simulink model "speed_pi_float"  (R2026b)
settings: Solver=FixedStepDiscrete  StopTime=0.01  FixedStep=0.0001
model workspace (MAT data in the model file):
  Iq_int_limit = 0.5
  Kaw_s = 0.08
  Ki_ASR = 1.44267798821
  Kp_ASR = 0.0180334748527
  Speed_loop_Iq_Limit = 1
  Ts = 0.0001
  Ts_ASR = 0.001
  v_ff_eps = 0.5
  v_over_eps = 3
  v_ref_zero_eps = 0
settings Model: Creator=lww  LastModifiedBy=lww

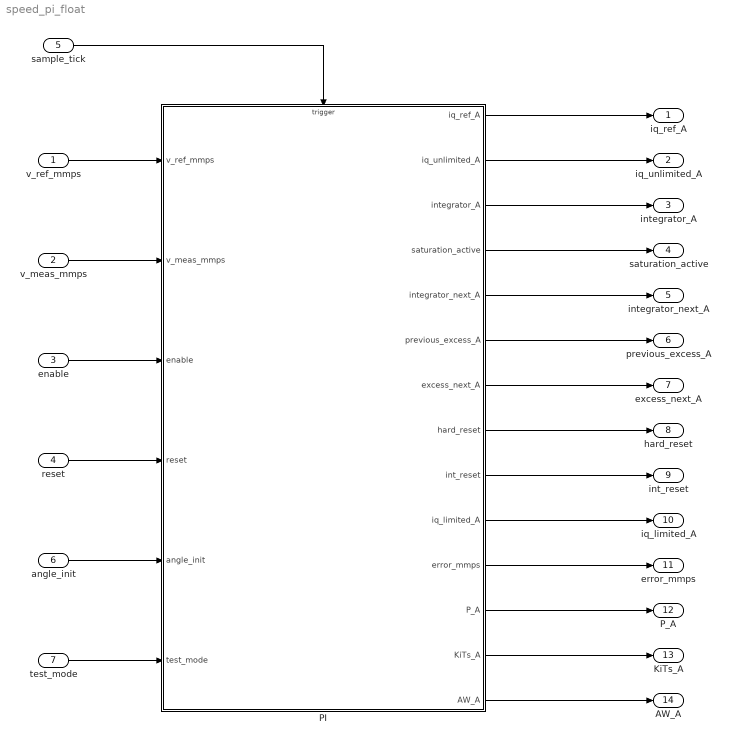
== system speed_pi_float ==
  v_ref_mmps : Inport
  v_meas_mmps : Inport  Port=2
  enable : Inport  Port=3
  reset : Inport  Port=4
  sample_tick : Inport  Port=5
  angle_init : Inport  Port=6
  test_mode : Inport  Port=7
  PI : Subsystem
  iq_ref_A : Outport
  iq_unlimited_A : Outport  Port=2
  integrator_A : Outport  Port=3
  saturation_active : Outport  Port=4
  integrator_next_A : Outport  Port=5
  previous_excess_A : Outport  Port=6
  excess_next_A : Outport  Port=7
  hard_reset : Outport  Port=8
  int_reset : Outport  Port=9
  iq_limited_A : Outport  Port=10
  error_mmps : Outport  Port=11
  P_A : Outport  Port=12
  KiTs_A : Outport  Port=13
  AW_A : Outport  Port=14
  wires:
  v_ref_mmps/1 -> PI/1(v_ref_mmps)
  sample_tick/1 -> PI/Trigger
  angle_init/1 -> PI/5(angle_init)
  v_meas_mmps/1 -> PI/2(v_meas_mmps)
  test_mode/1 -> PI/6(test_mode)
  enable/1 -> PI/3(enable)
  reset/1 -> PI/4(reset)
  PI/1(iq_ref_A) -> iq_ref_A/1
  PI/2(iq_unlimited_A) -> iq_unlimited_A/1
  PI/3(integrator_A) -> integrator_A/1
  PI/4(saturation_active) -> saturation_active/1
  PI/5(integrator_next_A) -> integrator_next_A/1
  PI/6(previous_excess_A) -> previous_excess_A/1
  PI/7(excess_next_A) -> excess_next_A/1
  PI/8(hard_reset) -> hard_reset/1
  PI/9(int_reset) -> int_reset/1
  PI/10(iq_limited_A) -> iq_limited_A/1
  PI/11(error_mmps) -> error_mmps/1
  PI/12(P_A) -> P_A/1
  PI/13(KiTs_A) -> KiTs_A/1
  PI/14(AW_A) -> AW_A/1

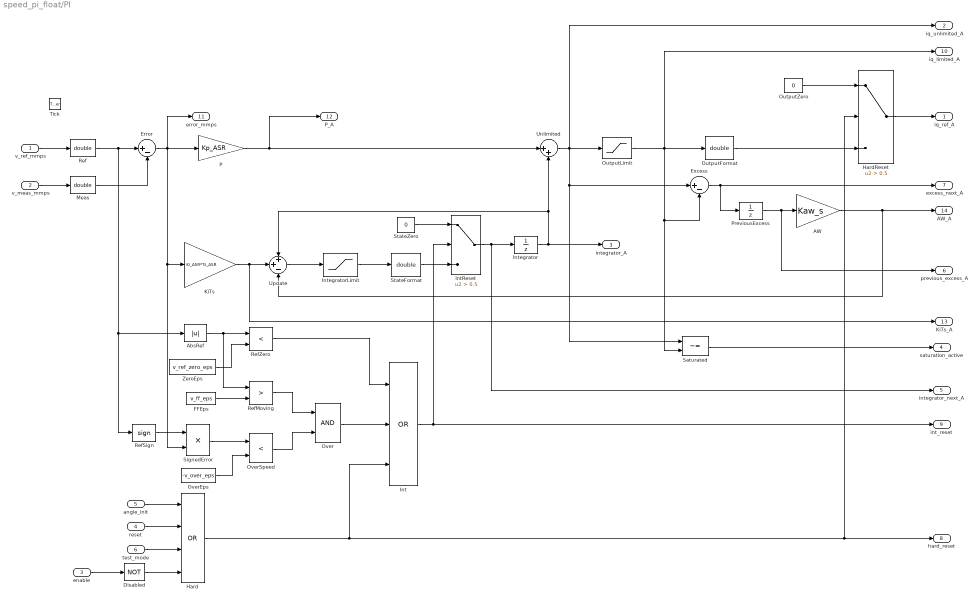
== system speed_pi_float/PI ==
  v_ref_mmps : Inport
  v_meas_mmps : Inport  Port=2
  enable : Inport  Port=3
  reset : Inport  Port=4
  angle_init : Inport  Port=5
  test_mode : Inport  Port=6
  Tick : TriggerPort  VariantControl=(inherit)
  AW : Gain  Gain=Kaw_s  ParamDataTypeStr=double  OutDataTypeStr=double  RndMeth=Convergent  SaturateOnIntegerOverflow=on
  AbsRef : Abs  RndMeth=Convergent
  Disabled : Logic  Operator=NOT  AllPortsSameDT=off  OutDataTypeStr=boolean
  Error : Sum  Inputs=|+-  OutDataTypeStr=double  AccumDataTypeStr=double  RndMeth=Convergent  SaturateOnIntegerOverflow=on
  Excess : Sum  Inputs=|+-  OutDataTypeStr=double  AccumDataTypeStr=double  RndMeth=Convergent  SaturateOnIntegerOverflow=on
  FFEps : Constant  Value=v_ff_eps  OutDataTypeStr=double
  Hard : Logic  Operator=OR  Inputs=4  AllPortsSameDT=off  OutDataTypeStr=boolean
  HardReset : Switch  Criteria=u2 > Threshold  Threshold=0.5  RndMeth=Convergent  InputSameDT=off
  Int : Logic  Operator=OR  Inputs=3  AllPortsSameDT=off  OutDataTypeStr=boolean
  IntReset : Switch  Criteria=u2 > Threshold  Threshold=0.5  RndMeth=Convergent  InputSameDT=off
  Integrator : UnitDelay  SampleTime=-1
  IntegratorLimit : Saturate  UpperLimit=Iq_int_limit  LowerLimit=-Iq_int_limit  RndMeth=Convergent
  KiTs : Gain  Gain=Ki_ASR*Ts_ASR  ParamDataTypeStr=double  OutDataTypeStr=double  RndMeth=Convergent  SaturateOnIntegerOverflow=on
  Meas : DataTypeConversion  OutDataTypeStr=double  RndMeth=Convergent
  OutputFormat : DataTypeConversion  OutDataTypeStr=double  RndMeth=Convergent
  OutputLimit : Saturate  UpperLimit=Speed_loop_Iq_Limit  LowerLimit=-Speed_loop_Iq_Limit  RndMeth=Convergent
  OutputZero : Constant  Value=0  OutDataTypeStr=double
  Over : Logic  AllPortsSameDT=off  OutDataTypeStr=boolean
  OverEps : Constant  Value=-v_over_eps  OutDataTypeStr=double
  OverSpeed : RelationalOperator  Operator=<  RndMeth=Convergent  InputSameDT=off
  P : Gain  Gain=Kp_ASR  ParamDataTypeStr=double  OutDataTypeStr=double  RndMeth=Convergent  SaturateOnIntegerOverflow=on
  PreviousExcess : UnitDelay  SampleTime=-1
  Ref : DataTypeConversion  OutDataTypeStr=double  RndMeth=Convergent
  RefMoving : RelationalOperator  Operator=>  RndMeth=Convergent  InputSameDT=off
  RefSign : Signum
  RefZero : RelationalOperator  Operator=<  RndMeth=Convergent  InputSameDT=off
  Saturated : RelationalOperator  Operator=~=  RndMeth=Convergent  InputSameDT=off
  SignedError : Product  OutDataTypeStr=double  RndMeth=Convergent  SaturateOnIntegerOverflow=on
  StateFormat : DataTypeConversion  OutDataTypeStr=double  RndMeth=Convergent
  StateZero : Constant  Value=0  OutDataTypeStr=double
  Unlimited : Sum  Inputs=|++  OutDataTypeStr=double  AccumDataTypeStr=double  RndMeth=Convergent  SaturateOnIntegerOverflow=on
  Update : Sum  Inputs=++-  OutDataTypeStr=double  AccumDataTypeStr=double  RndMeth=Convergent  SaturateOnIntegerOverflow=on
  ZeroEps : Constant  Value=v_ref_zero_eps  OutDataTypeStr=double
  iq_ref_A : Outport
  iq_unlimited_A : Outport  Port=2
  integrator_A : Outport  Port=3
  saturation_active : Outport  Port=4
  integrator_next_A : Outport  Port=5
  previous_excess_A : Outport  Port=6
  excess_next_A : Outport  Port=7
  hard_reset : Outport  Port=8
  int_reset : Outport  Port=9
  iq_limited_A : Outport  Port=10
  error_mmps : Outport  Port=11
  P_A : Outport  Port=12
  KiTs_A : Outport  Port=13
  AW_A : Outport  Port=14
  wires:
  v_ref_mmps/1 -> Ref/1
  v_meas_mmps/1 -> Meas/1
  enable/1 -> Disabled/1
  Integrator/1 -> integrator_A/1, Update/1, Unlimited/2
  RefMoving/1 -> Over/1
  Ref/1 -> RefSign/1, AbsRef/1, Error/1
  Excess/1 -> PreviousExcess/1, excess_next_A/1
  Error/1 -> P/1, KiTs/1, SignedError/2, error_mmps/1
  Meas/1 -> Error/2
  RefSign/1 -> SignedError/1
  P/1 -> Unlimited/1, P_A/1
  Disabled/1 -> Hard/4
  AbsRef/1 -> RefMoving/1, RefZero/1
  ZeroEps/1 -> RefZero/2
  Hard/1 -> hard_reset/1, HardReset/2, Int/3
  FFEps/1 -> RefMoving/2
  SignedError/1 -> OverSpeed/1
  OutputLimit/1 -> Excess/2, Saturated/2, iq_limited_A/1, OutputFormat/1
  OverSpeed/1 -> Over/2
  OverEps/1 -> OverSpeed/2
  KiTs/1 -> Update/2, KiTs_A/1
  test_mode/1 -> Hard/3
  angle_init/1 -> Hard/1
  reset/1 -> Hard/2
  Update/1 -> IntegratorLimit/1
  OutputZero/1 -> HardReset/1
  IntReset/1 -> Integrator/1, integrator_next_A/1
  IntegratorLimit/1 -> StateFormat/1
  HardReset/1 -> iq_ref_A/1
  Int/1 -> IntReset/2, int_reset/1
  StateZero/1 -> IntReset/1
  StateFormat/1 -> IntReset/3
  Unlimited/1 -> Saturated/1, Excess/1, iq_unlimited_A/1, OutputLimit/1
  OutputFormat/1 -> HardReset/3
  Saturated/1 -> saturation_active/1
  PreviousExcess/1 -> previous_excess_A/1, AW/1
  AW/1 -> AW_A/1, Update/3
  RefZero/1 -> Int/1
  Over/1 -> Int/2
